simulink model "separator"  (R2025b)
settings: Solver=VariableStepAuto  StartTime=0.0  StopTime=3000  MaxStep=1  RelTol=1e-3
undefined symbols (not defined in the file): Ki, Kp
libraries: simulink x3, slpidlib x1
settings Model: Creator=24A1EENB0065  LastModifiedBy=24A1EENB0065

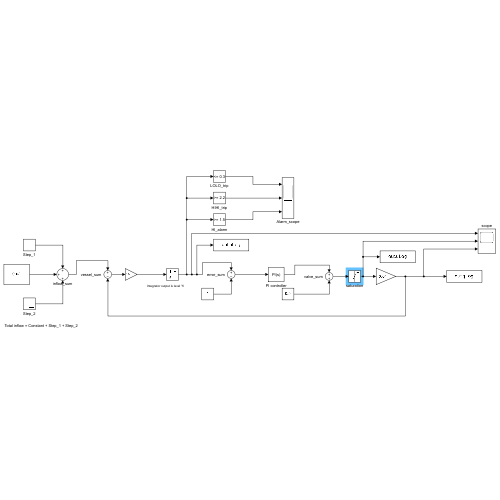
[thumbnail: Simulink's stored preview of the top-level diagram]
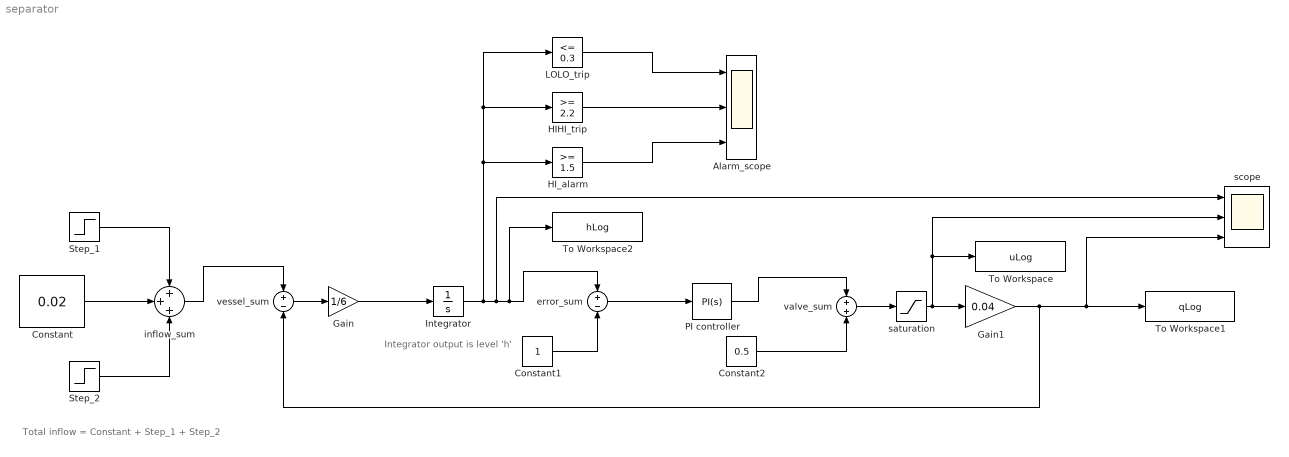
== system separator ==
  note: Integrator output is level 'h'
  note: Total inflow = Constant + Step_1 + Step_2
  Alarm_scope : Scope  NumInputPorts=3
      settings: ActiveDisplayYMinimum=-1  ActiveDisplayYMaximum=1
  Constant : Constant  Value=0.02
  Constant1 : Constant
  Constant2 : Constant  Value=0.5
  Gain : Gain  Gain=1/6
  Gain1 : Gain  Gain=0.04
  HIHI_trip : simulink/Logic and Bit Operations/Compare To Constant  relop=>=  const=2.2  OutDataTypeStr=boolean
  HI_alarm : simulink/Logic and Bit Operations/Compare To Constant  relop=>=  const=1.5  OutDataTypeStr=boolean
  Integrator : Integrator  InitialCondition=1  LimitOutput=on  UpperSaturationLimit=3  LowerSaturationLimit=0
  LOLO_trip : simulink/Logic and Bit Operations/Compare To Constant  relop=<=  const=0.3  OutDataTypeStr=boolean
  PI controller : slpidlib/PID Controller  Controller=PI  Form=Parallel  TimeDomain=Continuous-time  UseExternalTs=off  SampleTime=-1  IntegratorMethod=Forward Euler  FilterMethod=Forward Euler  ControllerParametersSource=internal  P=Kp  I=Ki  UseKiTs=off  D=0  UseExternalDerivativeSource=off  N=100  UseFilter=on  TunerSelectOption=Transfer Function Based (PID Tuner App)  InitialConditionSource=internal  InitialConditionForIntegrator=0  InitialConditionForFilter=0  DifferentiatorICPrevScaledInput=0  ExternalReset=none  TrackingMode=off  Kt=1  LimitOutput=off  SatLimitsSource=internal  UpperSaturationLimit=inf  LowerSaturationLimit=-inf  LinearizeAsGain=on  AntiWindupMode=none  Kb=1  LimitIntegrator=off  UpperIntegratorSaturationLimit=inf  LowerIntegratorSaturationLimit=-inf  POutMin=[]  POutMax=[]  IOutMin=[]  IOutMax=[]  DOutMin=[]  DOutMax=[]  NOutMin=[]  NOutMax=[]  SumOutMin=[]  SumOutMax=[]  SaturationOutMin=[]  SaturationOutMax=[]  PParamMin=[]  PParamMax=[]  IParamMin=[]  IParamMax=[]  DParamMin=[]  DParamMax=[]  NParamMin=[]  NParamMax=[]  KbParamMin=[]  KbParamMax=[]  KtParamMin=[]  KtParamMax=[]  KbOutMin=[]  KbOutMax=[]  KtOutMin=[]  KtOutMax=[]  IntegratorOutMin=[]  IntegratorOutMax=[]  FilterOutMin=[]  FilterOutMax=[]  SumI1OutMin=[]  SumI1OutMax=[]  SumI2OutMin=[]  SumI2OutMax=[]  SumI3OutMin=[]  SumI3OutMax=[]  SumI4OutMin=[]  SumI4OutMax=[]  SumDOutMin=[]  SumDOutMax=[]  DifferentiatorOutMin=[]  DifferentiatorOutMax=[]  FilterDiffOutCoefMin=[]  FilterDiffOutCoefMax=[]  ReciprocalOutMin=[]  ReciprocalOutMax=[]  SumDenOutMin=[]  SumDenOutMax=[]  SumNumOutMin=[]  SumNumOutMax=[]  DivideOutMin=[]  DivideOutMax=[]  UdiffTsProdOutMin=[]  UdiffTsProdOutMax=[]  NTsProdOutMin=[]  NTsProdOutMax=[]  UintegralTsProdOutMin=[]  UintegralTsProdOutMax=[]  UngainTsProdOutMin=[]  UngainTsProdOutMax=[]  ClampingZeroOutDataTypeStr=Inherit: Inherit via back propagation  ClampingZeroOutMin=[]  ClampingZeroOutMax=[]  FilterDenConstantOutDataTypeStr=Inherit: Inherit via back propagation  FilterDenConstantOutMin=[]  FilterDenConstantOutMax=[]  PCopyOutDataTypeStr=Inherit: Inherit via back propagation  PCopyOutMin=[]  PCopyOutMax=[]  NCopyOutDataTypeStr=Inherit: Inherit via back propagation  NCopyOutMin=[]  NCopyOutMax=[]  IntegratorContinuousStateAttributes=''  IntegratorStateMustResolveToSignalObject=off  IntegratorRTWStateStorageClass=Auto  FilterContinuousStateAttributes=''  FilterStateMustResolveToSignalObject=off  FilterRTWStateStorageClass=Auto  ParallelPVariant=InternalParameters  IdealPVariant=Disabled  IVariant=InternalParameters  DVariant=Disabled  IntegratorVariant=Continuous  SatVariant=Disabled  AWVariant=Passthrough  PCopyVariant=Disabled  TRVariant=Disabled  FdbkBlocksVariant=Forward  IdealPFdbkVariant=Disabled  SatFdbkVariant=Disabled  DerivativeFilterVariant=Disabled  NVariant=Disabled  NCopyVariant=Disabled_SignalSpec  FilterICVariant=Disabled  IntegratorICVariant=InternalICs  ExternalResetVariant=Disabled  TRSumVariant=Passthrough  SumFdbkVariant=Disabled  SumVariant=Sum_PI  TsampFilterVariant=InternalTs  TsampNgainVariant=Passthrough  TsampIntegralVariant=Disabled_SignalSpec  ExternalSaturationOutDataTypeStr=Inherit: Same as second input  DerivativeSourceVariant=Disabled  PreIntVariant=InternalPreInt
  Step_1 : Step  Time=100  After=0.015  SampleTime=0
  Step_2 : Step  Time=220  After=-0.015  SampleTime=0
  To Workspace : ToWorkspace  VariableName=uLog  SampleTime=-1
  To Workspace1 : ToWorkspace  VariableName=qLog  SampleTime=-1
  To Workspace2 : ToWorkspace  VariableName=hLog  SampleTime=-1
  error_sum : Sum  Inputs=+-
  inflow_sum : Sum  Inputs=+++
  saturation : Saturate  UpperLimit=1  LowerLimit=0
  scope : Scope  NumInputPorts=3
      settings: ActiveDisplayYMinimum=-0.47064813758533897  ActiveDisplayYMaximum=1.6236735061114289
  valve_sum : Sum
  vessel_sum : Sum  Inputs=+-
  wires:
  Step_1/1 -> inflow_sum/1
  Step_2/1 -> inflow_sum/3
  Constant/1 -> inflow_sum/2
  inflow_sum/1 -> vessel_sum/1
  vessel_sum/1 -> Gain/1
  Gain/1 -> Integrator/1
  Constant1/1 -> error_sum/2
  Integrator/1 -> LOLO_trip/1, HIHI_trip/1, HI_alarm/1, scope/1, error_sum/1, To Workspace2/1
  error_sum/1 -> PI controller/1
  PI controller/1 -> valve_sum/1
  Constant2/1 -> valve_sum/2
  valve_sum/1 -> saturation/1
  Gain1/1 -> scope/3, To Workspace1/1, vessel_sum/2
  saturation/1 -> Gain1/1, scope/2, To Workspace/1
  LOLO_trip/1 -> Alarm_scope/1
  HIHI_trip/1 -> Alarm_scope/2
  HI_alarm/1 -> Alarm_scope/3
